simulink model "model3_p_controller_hw"  (R2024b)
settings: Solver=FixedStepDiscrete  StartTime=0.0  StopTime=10  FixedStep=0.002  RelTol=1e-3  EnableMultiTasking=on
undefined symbols (not defined in the file or in its folder): HIL
libraries: quarc_library x5
settings Model: ExtModeTrigDuration=5000  Creator=hp  LastModifiedBy=hp
settings SolverCC: AlgebraicLoopSolver=TrustRegion  PositivePriorityOrder=on
settings DataIOCC: ReturnWorkspaceOutputs=off
settings DebuggingCC: UnconnectedInputMsg=warning  UnconnectedOutputMsg=warning  UnconnectedLineMsg=warning  ArithmeticOperatorsInVariantConditions=warning
settings ModelReferenceCC: EnableRefExpFcnMdlSchedulingChecks=on
settings SFSimCC: SimUseLocalCustomCode=off  CustomCodeUndefinedFunction=UseInterfaceOnly
settings RTWCC: Description=QUARC Win64 Target Using Toolchain  SystemTargetFile=quarc_win64.tlc  TemplateMakefile=quarc_default_tmf  RTWUseLocalCustomCode=off  Toolchain=QUARC win64 | nmake (64-bit Windows)  BuildConfiguration=Faster Runs  GPUComputeCapability=3.5
settings CodeAppCC: StateflowObjectComments=on
settings STFCustomTargetCC: TargetLangStandard=C99 (ISO)  ConcurrentExecutionCompliant=on  GRTInterface=on  UseToolchainInfoCompliant=on  SystemTargetFile=quarc_win64.tlc
settings GRTTargetCC: ParMdlRefBuildCompliant=off  CompOptLevelCompliant=off  CombineOutputUpdateFcns=off  MatFileLogging=off  CPPClassGenCompliant=off  GRTInterface=on  ExtMode=on  ExtModeMexFile=quarc_comm
settings ConfigComp: CovMetricSettings=dswe

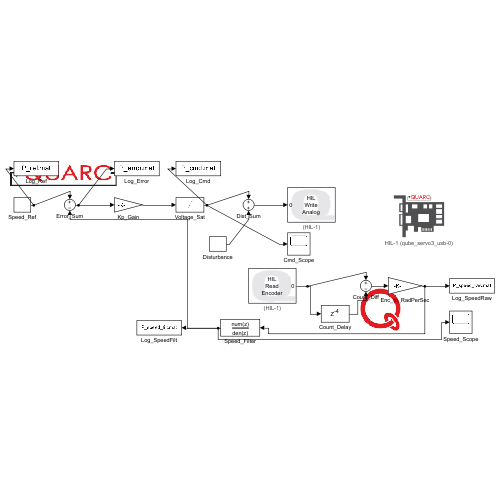
[thumbnail: Simulink's stored preview of the top-level diagram]
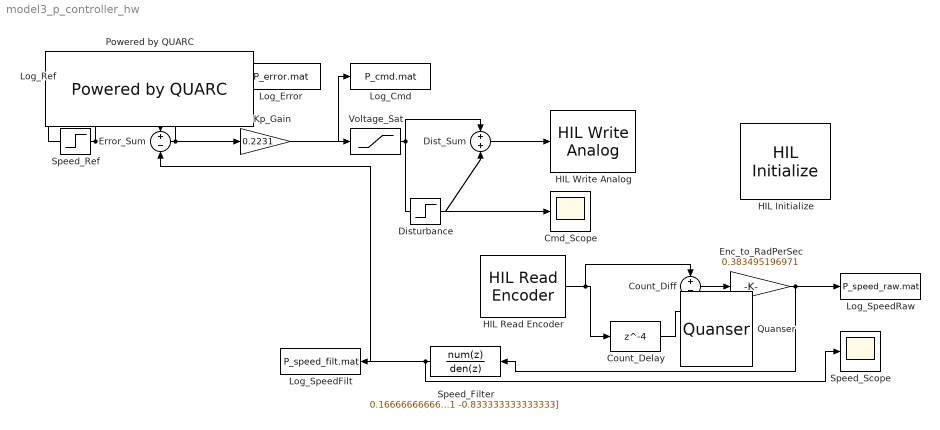
== system model3_p_controller_hw ==
  Cmd_Scope : Scope
  Count_Delay : Delay  DelayLength=4  InitialCondition=0  SampleTime=0.002
  Count_Diff : Sum  Inputs=+-
  Dist_Sum : Sum
  Disturbance : Step  Time=5  After=0.5  SampleTime=0
  Enc_to_RadPerSec : Gain  Gain=0.383495196971
  Error_Sum : Sum  Inputs=+-
  HIL Initialize : quarc_library/Data Acquisition/Generic/Configuration/HIL Initialize  object_name=HIL-1  board_type=qube_servo3_usb  board_number=0  board_options=""  exclusive=off  active=on  hardware_clocks=[0]  clock_modes=[]  initial_clock_frequencies=[]  set_clock_params_at_start=off  set_clock_params_at_switch_in=off  set_clock_frequencies_at_start=off  set_clock_frequencies_at_switch_in=off  analog_input_channels=[0]  analog_input_configurations=[]  analog_input_maximums=3  analog_input_minimums=-3  set_analog_input_params_at_start=off  set_analog_input_params_at_switch_in=off  analog_output_channels=[0]  analog_output_maximums=15  analog_output_minimums=-15  initial_analog_outputs=[0]  final_analog_outputs=[0]  watchdog_analog_outputs=0  set_analog_output_params_at_start=off  set_analog_output_params_at_switch_in=off  set_analog_outputs_at_start=on  set_analog_outputs_at_switch_in=off  set_analog_outputs_at_terminate=on  set_analog_outputs_at_switch_out=off  set_analog_outputs_on_watchdog=on  digital_input_channels=[]  digital_output_channels=[0]  digital_output_configuration=[]  initial_digital_outputs=[1]  final_digital_outputs=[0]  watchdog_digital_outputs=[0]  set_digital_output_params_at_start=off  set_digital_output_params_at_switch_in=off  set_digital_outputs_at_start=on  set_digital_outputs_at_switch_in=off  set_digital_outputs_at_terminate=on  set_digital_outputs_at_switch_out=off  set_digital_outputs_on_watchdog=on  encoder_channels=[0:1]  quadrature=[4]  encoder_filter_frequency=[]  initial_encoder_counts=[0]  set_encoder_params_at_start=off  set_encoder_params_at_switch_in=off  set_encoder_counts_at_start=on  set_encoder_counts_at_switch_in=off  pwm_channels=[]  pwm_modes=[0]  pwm_frequency=23195  pwm_configuration=[1]  pwm_alignment=[0]  pwm_polarity=[1]  pwm_leading_deadband=[0]  pwm_trailing_deadband=[0]  initial_pwm_outputs=[0]  final_pwm_outputs=[0]  watchdog_pwm_outputs=[]  set_pwm_params_at_start=off  set_pwm_params_at_switch_in=off  set_pwm_outputs_at_start=off  set_pwm_outputs_at_switch_in=off  set_pwm_outputs_at_terminate=off  set_pwm_outputs_at_switch_out=off  set_pwm_outputs_on_watchdog=off  other_output_channels=[11000:11002]  initial_other_outputs=[0 1 0]  final_other_outputs=[1 0 0]  watchdog_other_outputs=[0 0 1]  set_other_outputs_at_start=on  set_other_outputs_at_switch_in=off  set_other_outputs_at_terminate=on  set_other_outputs_at_switch_out=off  set_other_outputs_on_watchdog=on
  HIL Read Encoder : quarc_library/Data Acquisition/Generic/Immediate I//O/HIL Read Encoder  object_name=HIL-1  channels=0  sample_time=qc_get_step_size  active=on  vector_output=off  data_type_mode=Inherit via back propagation  data_type=double
  HIL Write Analog : quarc_library/Data Acquisition/Generic/Immediate I//O/HIL Write Analog  object_name=HIL-1  channels=0  sample_time=-1  active=off  vector_input=off
  Kp_Gain : Gain  Gain=0.2231
  Log_Cmd : ToFile  Filename=P_cmd.mat  MatrixName=P_cmd  SampleTime=0.002
  Log_Error : ToFile  Filename=P_error.mat  MatrixName=P_error  SampleTime=0.002
  Log_Ref : ToFile  Filename=P_ref.mat  MatrixName=P_ref  SampleTime=0.002
  Log_SpeedFilt : ToFile  Filename=P_speed_filt.mat  MatrixName=P_speed_filt  SampleTime=0.002
  Log_SpeedRaw : ToFile  Filename=P_speed_raw.mat  MatrixName=P_speed_raw  SampleTime=0.002
  Powered by QUARC : quarc_library/Logos/Powered by QUARC
  Quanser : quarc_library/Logos/Quanser
  Speed_Filter : DiscreteFilter  Numerator=0.166666666666667  Denominator=[1 -0.833333333333333]  SampleTime=0.002
  Speed_Ref : Step  After=50  SampleTime=0
  Speed_Scope : Scope
  Voltage_Sat : Saturate  UpperLimit=10  LowerLimit=-10
  wires:
  Speed_Ref/1 -> Error_Sum/1, Log_Ref/1
  Error_Sum/1 -> Kp_Gain/1, Log_Error/1
  Kp_Gain/1 -> Voltage_Sat/1
  Voltage_Sat/1 -> Dist_Sum/1, Log_Cmd/1, Cmd_Scope/1
  Disturbance/1 -> Dist_Sum/2
  Dist_Sum/1 -> HIL Write Analog/1
  HIL Read Encoder/1 -> Count_Delay/1, Count_Diff/1
  Count_Delay/1 -> Count_Diff/2
  Count_Diff/1 -> Enc_to_RadPerSec/1
  Enc_to_RadPerSec/1 -> Speed_Filter/1, Log_SpeedRaw/1
  Speed_Filter/1 -> Error_Sum/2, Log_SpeedFilt/1, Speed_Scope/1
